simulink model "OSWEC"  (R2020b)
settings: Solver=ode4  StartTime=0  StopTime=600  FixedStep=0.01  MaxStep=0.01  RelTol=1e-3  EnableMultiTasking=on
values from neighbouring files (symbols this model uses):
  bemDirections = sort(unique(bemDirections))    [runCases.m]    (also in wecSimInputFile.m = -30:0.25:30)
  waves = waveClass('regular')    [wecSimInputFile.m]
undefined symbols (not defined in the file or in its folder): body, constraint, geometry, hydroData, pto
libraries: WECSim_Lib_Body_Elements x2, WECSim_Lib_Constraints x1, WECSim_Lib_Frames x1, WECSim_Lib_PTOs x1
settings Model: Creator=mlawson  LastModifiedBy=akeeste
settings SolverCC: ZeroCrossControl=DisableAll  AlgebraicLoopSolver=LineSearch  AutoInsertRateTranBlk=on
settings DataIOCC: SaveFormat=Array  SaveOutput=off  SaveTime=off  ReturnWorkspaceOutputs=off
settings OptimizationCC: LifeSpan=inf  SimCompilerOptimization=on
settings DebuggingCC: MergeDetectMultiDrivingBlocksExec=none  SolverPrmCheckMsg=warning  AllowSymbolicDim=off  StateNameClashWarn=warning  SFUnexpectedBacktrackingDiag=warning  SFNoUnconditionalDefaultTransitionDiag=warning  SFExecutionAtInitializationDiag=none  ArithmeticOperatorsInVariantConditions=warning
settings HardwareCC: ProdBitPerPointer=32  ProdBitPerSizeT=32  ProdBitPerPtrDiffT=32  ProdLargestAtomicFloat=None  ProdIntDivRoundTo=Undefined  ProdEndianess=Unspecified  ProdWordSize=32  ProdHWDeviceType=32-bit Generic
settings ModelReferenceCC: PropagateSignalLabelsOutOfModel=off
settings SFSimCC: SimUseLocalCustomCode=off  CustomCodeUndefinedFunction=UseInterfaceOnly
settings RTWCC: RTWUseLocalCustomCode=off
settings CodeAppCC: StateflowObjectComments=on
settings GRTTargetCC: TargetLangStandard=C89/C90 (ANSI)
settings ConfigComp: CovMetricSettings=dw  CovSaveCumulativeToWorkspaceVar=on  CovSaveSingleToWorkspaceVar=on  CovExternalEMLEnable=off  CovSFcnEnable=off
settings SimscapeCC: SimscapeNormalizeSystem=off
settings ConfigurationSet: Description=SimMechanics 2G
settings ExplorerConfigSet: InternalSimMechanicsExplorerSettings="<ExplorerConfiguration><canonicalview>default</canonicalview><TilePanel><TileInfo><Tiles Columns=\"1\" Count=\"1\" Rows=\"1\"><Column Left=\"2\" Weight=\"1\"/><Column Left=\"1335\"/><Row Top=\"2\" Weight=\"1\"/><Row Top=\"911\"/><Tile Height=\"1\" Width=\"1\" X=\"0\" Y=\"0\"/></Tiles></TileInfo><SceneInfo><SceneViewer><BGColor><R>0.60000002384185791</R><G>0.60000002384185791</G><B>0.60000002384185791</B></BGColor><Camera><Position><X>365.37645888990272</X><Y>-369.82486814446582</Y><Z>359.64809521743916</Z></Position><Center><X>-6.7351450971904585</X><Y>2.2867358426280204</Y><Z>-12.463508769654169</Z></Center><Up><X>-0.40824829046386307</X><Y>0.40824829046386307</Y><Z>0.81649658092772615</Z></Up><Left>-57.820127362122818</Left><Right>57.820127362122818</Right><Bottom>-38.308817187253304</Bottom><Top>38.308817187253304</Top></Camera></SceneViewer></SceneInfo></TilePanel></ExplorerConfiguration>"

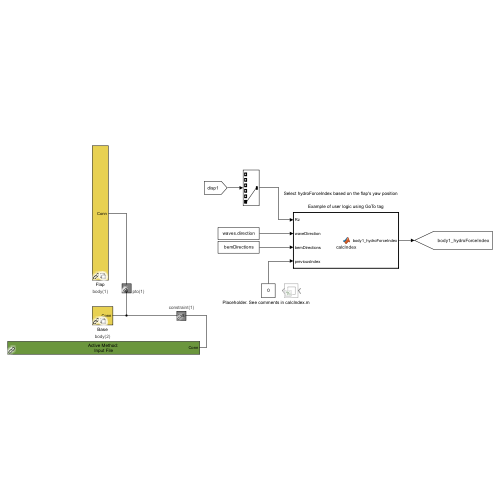
[thumbnail: Simulink's stored preview of the top-level diagram]
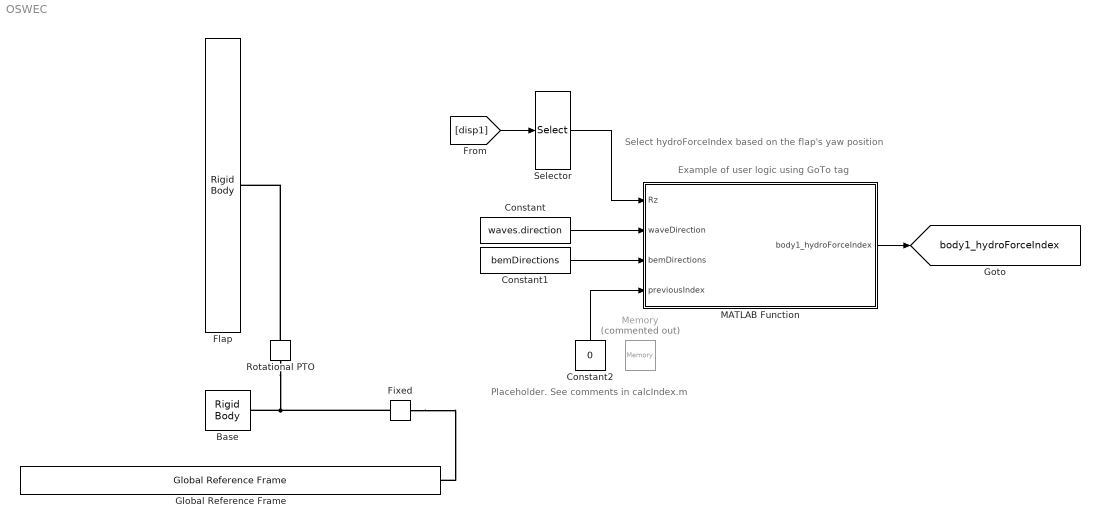
== system OSWEC ==
  note: Placeholder. See comments in calcIndex.m
  note: Example of user logic using GoTo tag
  note: Select hydroForceIndex based on the flap's yaw position
  Base : WECSim_Lib_Body_Elements/Rigid Body  body=body(2)  h5File=hydroData/*.h5  geometryFile=geometry/*.stl  mass=0  inertia=0 0 0  inertiaProducts=0 0 0  nonHydro=0  nonlinearHydro=0  centerGravity=0 0 0  centerBuoyancy=0 0 0  dof=6  volume=0  displacement=0 0 0  axis=0 1 0  angle=0  option=0  cd=0 0 0  ca=0 0 0  area=0 0 0  VME=0  rgME=0 0 0  z=0 0 1
  Constant : Constant  Value=waves.direction
  Constant1 : Constant  Value=bemDirections
  Constant2 : Constant  Value=0
  Fixed : WECSim_Lib_Constraints/Fixed  constraint=constraint(1)  loc="0  0  0"  displacement=0 0 0  y=0 1 0  z=0 0 1  upperLimitSpecify=off  upperLimitBound=0  upperLimitTransitionRegionWidth=0  upperLimitStiffness=0  upperLimitDamping=0  lowerLimitSpecify=off  lowerLimitBound=0  lowerLimitTransitionRegionWidth=0  lowerLimitStiffness=0  lowerLimitDamping=0
      settings: AttributesFormatString=%<constraint>
  Flap : WECSim_Lib_Body_Elements/Rigid Body  body=body(1)  h5File=hydroData/*.h5  geometryFile=geometry/*.stl  mass=0  inertia=0 0 0  inertiaProducts=0 0 0  nonHydro=0  nonlinearHydro=0  centerGravity=0 0 0  centerBuoyancy=0 0 0  dof=6  volume=0  displacement=0 0 0  axis=0 1 0  angle=0  option=0  cd=0 0 0  ca=0 0 0  area=0 0 0  VME=0  rgME=0 0 0  z=0 0 1
  Global Reference Frame : WECSim_Lib_Frames/Global Reference Frame  waves=waves  simu=simu  InputMethod=Input File  InputFile=wecSimInputFile.m  mode=normal  explorer=off  solver=ode4  startTime=0  rampTime=100  endTime=400  dt=0.1  cicEndTime=60  stateSpace=0  WaveClass=regular  height=2.5  period=8  elevationFile=NOT DEFINED  spectrumFile=NOT DEFINED  direction=0  spread=1  spectrumType=NOT DEFINED  phaseSeed=0  option=EqualEnergy
  MATLAB Function : MATLAB Function  TreatAsAtomicUnit=on
  Memory : Memory  Commented=on  InitialCondition=body(1).variableHydro.hydroForceIndexInitial
  Rotational PTO : WECSim_Lib_PTOs/Rotational PTO  pto=pto(1)  loc="0  0  0"  stiffness=0  damping=0  equilibriumPosition=0  pretension=0  displacement=0 0 0  y=0 1 0  z=0 0 1  upperLimitSpecify=off  upperLimitBound=0  upperLimitTransitionRegionWidth=0  upperLimitStiffness=0  upperLimitDamping=0  lowerLimitSpecify=off  lowerLimitBound=0  lowerLimitTransitionRegionWidth=0  lowerLimitStiffness=0  lowerLimitDamping=0
      settings: AttributesFormatString=%<pto>
  Selector : Selector  InputPortWidth=6  IndexOptions=Index vector (dialog)  Indices=[6]  OutputSizes=1
  tag scope: body1_hydroForceIndex=global
  wires:
  Selector/1 -> MATLAB Function/1(Rz)
  MATLAB Function/1(body1_hydroForceIndex) -> [body1_hydroForceIndex]
  [disp1] -> Selector/1
  Constant/1 -> MATLAB Function/2(waveDirection)
  Constant1/1 -> MATLAB Function/3(bemDirections)
  Constant2/1 -> MATLAB Function/4(previousIndex)
  connections:
  Fixed/LConn1 -- Global Reference Frame/RConn1
  Fixed/RConn1 -- Rotational PTO/LConn1 -- Base/RConn1
  Rotational PTO/RConn1 -- Flap/RConn1

== matlab function OSWEC/MATLAB Function ==
  data: Rz input; waveDirection input; bemDirections input; body1_hydroForceIndex output; previousIndex input
function body1_hydroForceIndex  = calcIndex(Rz, waveDirection, bemDirections, previousIndex)

body1_hydroForceIndex  = calcIndex(Rz, waveDirection, bemDirections, previousIndex);

end
